simulink model "dc_motor_simscape_open_loop"  (R2024b)
settings: Solver=ode15s  StartTime=0.0  StopTime=5  RelTol=1e-3  AbsTol=1e-3
libraries: fl_lib x10, nesl_utility x4
settings Model: Creator=Taha  LastModifiedBy=Taha
settings SolverCC: AutoScaleAbsTol=off  AlgebraicLoopSolver=TrustRegion  MaxZcPerStep=1
settings DebuggingCC: UnconnectedInputMsg=warning  UnconnectedOutputMsg=warning  UnconnectedLineMsg=warning  SymbolicDimsDataTypeCodeGenerationDiagnostic=none
settings ModelReferenceCC: EnableRefExpFcnMdlSchedulingChecks=on
settings SFSimCC: CustomCodeUndefinedFunction=UseInterfaceOnly
settings RTWCC: GPUComputeCapability=3.5  DLArmComputeVersion=19.05
settings SimscapeCC: SimscapeLogType=all  SimscapeLogSimulationStatistics=on  SimscapeLogDataHistory=10000

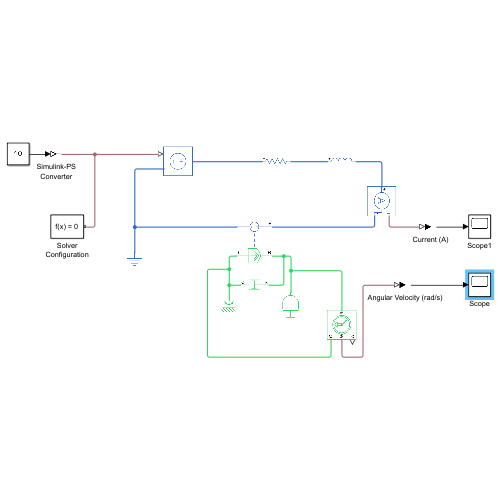
[thumbnail: Simulink's stored preview of the top-level diagram]
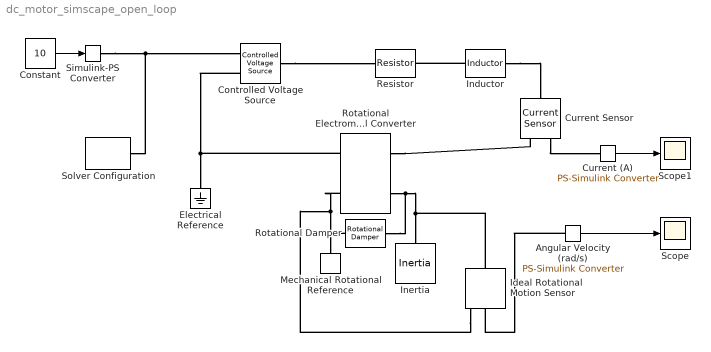
== system dc_motor_simscape_open_loop ==
  Angular Velocity (rad/s) : nesl_utility/PS-Simulink Converter  PhysicalDomain=network_engine_domain  SubClassName=ps_output  LeftPortType=input  RightPortType=output  PseudoPeriodic=off  Frequencies=[]  VectorFormat=inherit  Unit=rad/s  AffineConversion=off
  Constant : Constant  Value=10
  Controlled Voltage Source : fl_lib/Electrical/Electrical Sources/Controlled Voltage Source
  Current (A) : nesl_utility/PS-Simulink Converter  PhysicalDomain=network_engine_domain  SubClassName=ps_output  LeftPortType=input  RightPortType=output  PseudoPeriodic=off  Frequencies=[]  VectorFormat=inherit  Unit=A  AffineConversion=off
  Current Sensor : fl_lib/Electrical/Electrical Sensors/Current Sensor
  Electrical Reference : fl_lib/Electrical/Electrical Elements/Electrical Reference
  Ideal Rotational Motion Sensor : fl_lib/Mechanical/Mechanical Sensors/Ideal Rotational Motion Sensor  reference=foundation.enum.MeasurementReference.difference  acceleration_port=false  velocity_port=true  position_port=true  wrap_angle=false  offset=0 rad
  Inductor : fl_lib/Electrical/Electrical Elements/Inductor  l=0.5 H  r=0 Ohm  g=1e-9 1/Ohm  i_specify=off  i_priority=None  i=0 A  i_nominal_specify=off  i_nominal_value=1  i_nominal_unit=A  v_specify=off  v_priority=None  v=0 V  v_nominal_specify=off  v_nominal_value=1  v_nominal_unit=V  i_L_specify=off  i_L_priority=High  i_L=0 A  i_L_nominal_specify=off  i_L_nominal_value=1  i_L_nominal_unit=A
  Inertia : fl_lib/Mechanical/Rotational Elements/Inertia  inertia=0.01 kg*m^2  num_ports=foundation.enum.numPorts2.one  w_specify=off  w_priority=High  w=0 rad/s  w_nominal_specify=off  w_nominal_value=1  w_nominal_unit=rad/s  t_specify=off  t_priority=None  t=0 N*m  t_nominal_specify=off  t_nominal_value=1  t_nominal_unit=N*m
  Mechanical Rotational Reference : fl_lib/Mechanical/Rotational Elements/Mechanical Rotational Reference
  Resistor : fl_lib/Electrical/Electrical Elements/Resistor  R=1 Ohm  i_specify=off  i_priority=None  i=0 A  i_nominal_specify=off  i_nominal_value=1  i_nominal_unit=A  v_specify=off  v_priority=None  v=0 V  v_nominal_specify=off  v_nominal_value=1  v_nominal_unit=V
  Rotational Electromechanical Converter : fl_lib/Electrical/Electrical Elements/Rotational Electromechanical Converter  K=0.01 V*s/rad  i_specify=off  i_priority=None  i=0 A  i_nominal_specify=off  i_nominal_value=1  i_nominal_unit=A  v_specify=off  v_priority=None  v=0 V  v_nominal_specify=off  v_nominal_value=1  v_nominal_unit=V  t_specify=off  t_priority=None  t=0 N*m  t_nominal_specify=off  t_nominal_value=1  t_nominal_unit=N*m  w_specify=off  w_priority=None  w=0 rad/s  w_nominal_specify=off  w_nominal_value=1  w_nominal_unit=rad/s
  Rotational Damper : fl_lib/Mechanical/Rotational Elements/Rotational Damper  D=0.1 N*m*s/rad  w_specify=off  w_priority=None  w=0 rad/s  w_nominal_specify=off  w_nominal_value=1  w_nominal_unit=rad/s  t_specify=off  t_priority=None  t=0 N*m  t_nominal_specify=off  t_nominal_value=1  t_nominal_unit=N*m
  Scope : Scope
  Scope1 : Scope
  Simulink-PS Converter : nesl_utility/Simulink-PS Converter  PhysicalDomain=network_engine_domain  SubClassName=ps_input  LeftPortType=input  RightPortType=output  PseudoPeriodic=off  Frequencies=[]  NoiseDistribution=none  NoiseParameters=[]  Unit=1  AffineConversion=off  FilteringAndDerivatives=provide  SimscapeFilterOrder=1  InputFilterTimeConstant=0.001  UdotUserProvided=0
  Solver Configuration : nesl_utility/Solver Configuration  PhysicalDomain=network_engine_domain  SubClassName=solver  LeftPortType=input  RightPortType=generic  Tones=[]  Harmonics=[]  SimulateNoise=off  Profile=off  UseLocalSampling=off  EnableSwitchedLinearOptims=on  FrequencyDomain=off  UseCCode=off  RelTol=0.001  AbsTol=1e-06  MinStep=1e-09  ToWorkspace=off  RevertToSquareIcSolve=off  NumHomotopyIterations=100  PhasorMode=off  PhasorModeNumHarmonics=1  ConsistencySolver=NEWTON_XTOL_AFTER_FTOL  IndexReductionMethod=DerivativeReplacement  DoDC=off  ResidualTolerance=1e-09  ConsistencyTolSource=GLOBAL  ConsistencyAbsTol=0.001  ConsistencyRelTol=0.001  ConsistencyTolFactor=0.001  UseLocalSolver=off  LocalSolverChoice=NE_BACKWARD_EULER_ADVANCER  ResolveIndetEquations=on  FunctionEvalNumThread=1  LocalSolverSampleTime=0.001  DoFixedCost=off  MaxNonlinIter=3  MaxModeIter=2  ComputeImpulses=off  ImpulseIterations=2  LinearAlgebra=auto  LinearAlgebraNumThread=0  EquationFormulation=NE_TIME_EF  DelaysMemoryBudget=1024  AutomaticFiltering=on  FilteringTimeConstant=0.001  PartitionStorageMethod=AS_NEEDED  PartitionMemoryBudget=1024  PartitionMethod=ROBUST  MultibodyUseLocalSolver=off  MultibodyLocalSolverChoice=ODE1  MultibodyLocalSolverSampleTime=0.001
  wires:
  Angular Velocity (rad/s)/1 -> Scope/1
  Constant/1 -> Simulink-PS Converter/1
  Current (A)/1 -> Scope1/1
  connections:
  Controlled Voltage Source/LConn1 -- Resistor/LConn1
  Inductor/LConn1 -- Resistor/RConn1
  Simulink-PS Converter/RConn1 -- Solver Configuration/RConn1 -- Controlled Voltage Source/RConn1
  Rotational Electromechanical Converter/LConn2 -- Rotational Damper/LConn1 -- Ideal Rotational Motion Sensor/LConn1 -- Inertia/LConn1
  Rotational Electromechanical Converter/RConn2 -- Ideal Rotational Motion Sensor/RConn1 -- Rotational Damper/RConn1 -- Mechanical Rotational Reference/LConn1
  Angular Velocity (rad/s)/LConn1 -- Ideal Rotational Motion Sensor/RConn2
  Controlled Voltage Source/RConn2 -- Rotational Electromechanical Converter/RConn1 -- Electrical Reference/LConn1
  Inductor/RConn1 -- Current Sensor/LConn1
  Current Sensor/RConn1 -- Current (A)/LConn1
  Rotational Electromechanical Converter/LConn1 -- Current Sensor/RConn2
